simulink model "ex_slides16_30_rotor_bars"  (R2026b)
settings: Solver=ode23t  StopTime=0.04  MaxStep=1e-4  RelTol=1e-5
libraries: asm_blocks_lib x6
settings Model: Creator=fsbb  LastModifiedBy=fsbb

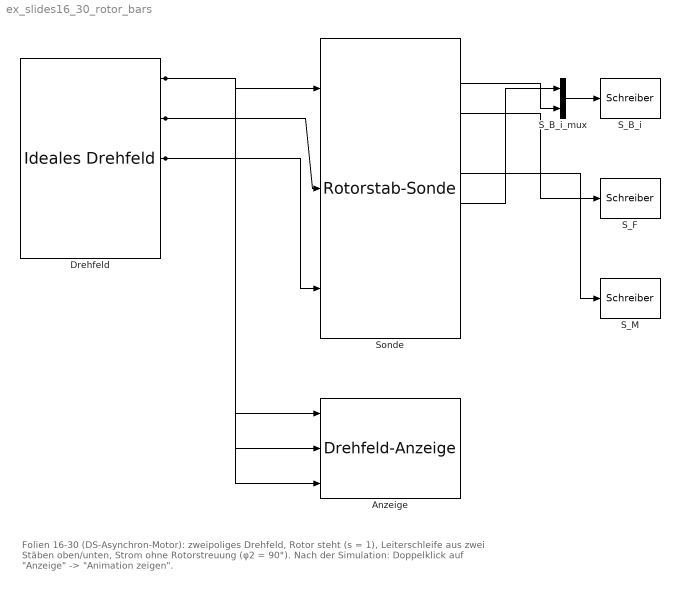
== system ex_slides16_30_rotor_bars ==
  note: Folien 16-30 (DS-Asynchron-Motor): zweipoliges Drehfeld, Rotor steht (s = 1), Leiterschleife aus zwei Stäben oben/unten, Strom ohne Rotorstreuung (φ2 = 90°). Nach der Simulation: Doppelklick auf "Anzeige" -> "Animation zeigen".
  Anzeige : asm_blocks_lib/Didaktik/Drehfeld-Anzeige  Tag=asmlib:field_display  view_frame=rotorfest  image_orientation=wie Folien (U1 oben, Feld im Uhrzeigersinn)  decomposition=on  change_vector=on  force_arrows=on  all_bars=on  slow_motion=0.01  N2=2  p=1  l=0.15  r=0.06  N1xi1=144  bar1_angle=-90
  Drehfeld : asm_blocks_lib/Didaktik/Ideales Drehfeld  Tag=asmlib:ideal_field  Bhat=0.8  f1=50  p=1  s=1  l=0.15  r=0.06  N1xi1=144  N2=2  R2_S=0.000318664  L2s_S=5.0717e-06  phi2_mode=fest  phi2_fix=90
  S_B_i : asm_blocks_lib/Messgeräte/Schreiber  Tag=asmlib:recorder  title_text=B⊥ und Strom Stab 1
  S_B_i_mux : Mux  Inputs=2
  S_F : asm_blocks_lib/Messgeräte/Schreiber  Tag=asmlib:recorder  title_text=Kraft Stab 1 und 2
  S_M : asm_blocks_lib/Messgeräte/Schreiber  Tag=asmlib:recorder  title_text=Moment der Schleife
  Sonde : asm_blocks_lib/Didaktik/Rotorstab-Sonde  Tag=asmlib:rotor_bar_probe  k1=1  k2=2  N2=2  p=1  l=0.15  r=0.06  N1xi1=144  bar1_angle=-90  convention=wie Folien (Strom aus der Zeichenebene positiv)
  wires:
  Drehfeld/1 -> Sonde/1, Anzeige/1
  Drehfeld/2 -> Sonde/2, Anzeige/2
  Drehfeld/3 -> Sonde/3, Anzeige/3
  Sonde/6 -> S_B_i_mux/1
  Sonde/2 -> S_B_i_mux/2
  S_B_i_mux/1 -> S_B_i/1
  Sonde/3 -> S_F/1
  Sonde/5 -> S_M/1
